simulink model "single_phase_afe"  (R2026b)
settings: Solver=ode23tb  StopTime=param.sim.simlength  FixedStep=param.sim.tc  MaxStep=param.glb_time.tc
values from neighbouring files (symbols this model uses):
  param = struct()    [init_model.m]
undefined symbols (not defined in the file or in its folder): magnitude
libraries: fl_lib x201, nesl_utility x108, igbt_simple_2th_lib x8, single_phase_pwm_modulator x2, dq_vector_pi x2, phase_shift_filter_ccaller x2, pi_ctrl x2, discrete_time_low_pass_filter x2, lithium_ion_battery x1, dclink_for_two_levels x1, three_phase_voltage_with_frt_emulator x1, simulink x1
(part 1 of 7)
settings Model: SimulationMode=accelerator  Creator=LTNBDA  LastModifiedBy=dbagn
settings SolverCC: AutoInsertRateTranBlk=on  SolverResetMethod=Robust  ZeroCrossAlgorithm=Adaptive  ZeroCrossControl=DisableAll
settings DataIOCC: DSMLogging=off  LimitDataPoints=on  MaxDataPoints=1  ReturnWorkspaceOutputs=off  SaveFormat=Array  SaveOutput=off  SaveTime=off  SignalLogging=off  SignalLoggingSaveFormat=ModelDataLogs
settings OptimizationCC: EfficientMapNaN2IntZero=off  LifeSpan=inf  MemsetInitFltsAndDblsToZero=off
settings DebuggingCC: ArithmeticOperatorsInVariantConditions=warning  FcnCallInpInsideContextMsg=warning  IgnoredZcDiagnostic=none  MergeDetectMultiDrivingBlocksExec=none  MultiTaskCondExecSysMsg=none  MultiTaskDSMMsg=warning  MultiTaskRateTransMsg=warning  SFNoUnconditionalDefaultTransitionDiag=warning  SFUnexpectedBacktrackingDiag=warning  SaveWithParameterizedLinksMsg=none  SignalResolutionControl=TryResolveAllWithWarning  SolverPrmCheckMsg=warning  StateNameClashWarn=warning
settings HardwareCC: ProdEndianess=Unspecified  ProdEqTarget=off  ProdHWDeviceType=Generic->64-bit Embedded Processor (LP64)  ProdIntDivRoundTo=Undefined  ProdLargestAtomicFloat=None  TargetEndianess=LittleEndian  TargetHWDeviceType=MATLAB Host  TargetIntDivRoundTo=Zero  TargetLongLongMode=on
settings ModelReferenceCC: PropagateSignalLabelsOutOfModel=off
settings SFSimCC: CustomCodeUndefinedFunction=UseInterfaceOnly  SimUseLocalCustomCode=off
settings SFSimCC: SimCustomHeaderCode=|
  | #include "phase_shift_flt_simulink.h"
  | #include "sv_pwm.h"
  | #include "rpi.h"
  | #include "rpi_simulink.h"
  | #include "first_harmonic_tracker.h"
  | #include "dqvector_pi.h"
  | #include "dqvector_pi_simulink.h"
  | #include "sv_pwm_simulink.h"
  | #include "dqpll_grid.h"
  | #include "first_harmonic_tracker_simulink.h"
  | #include "dqpll_grid_simulink.h"
  | #include "phase_shift_flt.h"
  | #include "math_f.h"
  | #include "linear_double_integrator_observer_simulink.h"
  | #include "linear_double_integrator_observer.h"
  | #include "sogi_flt_simulink.h"
  | #include "sogi_flt.h"
settings SFSimCC: SimUserIncludeDirs=|
  | include
  | src
settings SFSimCC: SimUserSources=|
  | "rpi.c"
  | "rpi_simulink.c"
  | "dqvector_pi_simulink.c"
  | "dqvector_pi.c"
  | "sv_pwm_simulink.c"
  | "sv_pwm.c"
  | "first_harmonic_tracker_simulink.c"
  | "first_harmonic_tracker.c"
  | "dqpll_grid_simulink.c"
  | "dqpll_grid.c"
  | "phase_shift_flt_simulink.c"
  | "phase_shift_flt.c"
  | "linear_double_integrator_observer_simulink.c"
  | "linear_double_integrator_observer.c"
  | "sogi_flt_simulink.c"
  | "sogi_flt.c"
settings RTWCC: RTWUseLocalCustomCode=off
settings CodeAppCC: StateflowObjectComments=on
settings GRTTargetCC: CombineOutputUpdateFcns=off  GRTInterface=on  TargetLangStandard=C89/C90 (ANSI)
settings ConfigComp: CovExternalEMLEnable=off  CovSaveCumulativeToWorkspaceVar=on  CovSaveSingleToWorkspaceVar=on
settings SimscapeCC: SimscapeNormalizeSystem=off  SimscapeUseEnergyAccounting=off

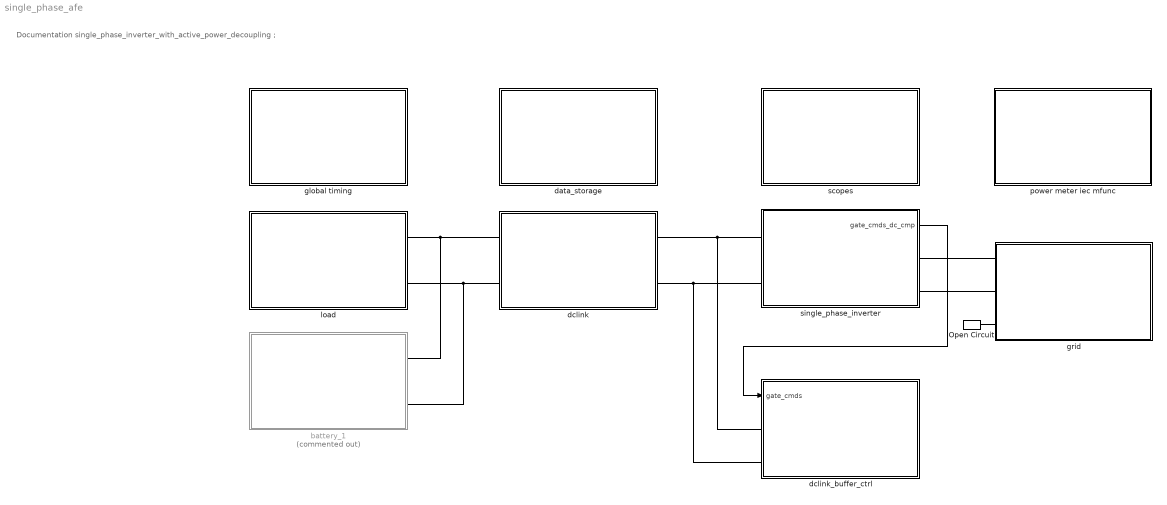
== system single_phase_afe ==
  note: Documentation
      | single_phase_inverter_with_active_power_decoupling ;
  Open Circuit : fl_lib/Electrical/Electrical Elements/Open Circuit  v_specify=off  v_priority=None  v=0 V  v_nominal_specify=off  v_nominal_value=1  v_nominal_unit=V
  battery_1 : Subsystem  Commented=on
  data_storage : Subsystem
  dclink : Subsystem
  dclink_buffer_ctrl : Subsystem
  global timing : Subsystem
  grid : Subsystem
  load : Subsystem
  power meter iec mfunc : Subsystem
  scopes : Subsystem
  single_phase_inverter : Subsystem
  wires:
  single_phase_inverter/1(gate_cmds_dc_cmp) -> dclink_buffer_ctrl/1(gate_cmds)
  connections:
  dclink/RConn2 -- dclink_buffer_ctrl/LConn2 -- single_phase_inverter/LConn2
  dclink/RConn1 -- dclink_buffer_ctrl/LConn1 -- single_phase_inverter/LConn1
  load/LConn2 -- battery_1/RConn2 -- dclink/LConn2
  load/LConn1 -- battery_1/RConn1 -- dclink/LConn1
  grid/RConn1 -- single_phase_inverter/RConn1
  grid/RConn2 -- single_phase_inverter/RConn2
  Open Circuit/LConn1 -- grid/RConn3

== system single_phase_afe/battery_1 ==
  To Workspace14 : ToWorkspace  VariableName=battery_1_data_sim  SampleTime=param.glb_time.tc
      settings: MaxDataPoints=param.glb_time.Nc  Decimation=param.glb_time.decimation_tc
  lithium ion battery : Scope
      settings: ActiveDisplayYMinimum=1112.6382819704118  ActiveDisplayYMaximum=1354.3206561925681  DataLoggingVariableName=ScopeData3
  lithium_ion_battery : lithium_ion_battery/lithium_ion_battery  Q=param.battery.pack_1.Q  number_of_cells=param.battery.pack_1.number_of_cells  E_1=param.battery.pack_1.E_1  E0=param.battery.pack_1.E0  E1=param.battery.pack_1.E1  E2=param.battery.pack_1.E2  E3=param.battery.pack_1.E3  Elog=param.battery.pack_1.Elog  R0=param.battery.pack_1.R0  R1=param.battery.pack_1.R1  C1=param.battery.pack_1.C1  M=param.battery.pack_1.M  alpha=param.battery.pack_1.alpha  soc_init=param.battery.pack_1.soc_init  ts_battery=param.glb_time.ts_dab  q1Kalman=param.battery.pack_1.q1Kalman  q2Kalman=param.battery.pack_1.q2Kalman  q3Kalman=param.battery.pack_1.q3Kalman  rKalman=param.battery.pack_1.rKalman  tc=param.glb_time.tc  enable_white_noise_m=0  battery_voltage_init_m=param.battery.nominal_battery_voltage_1
  single_phase_ui_measure : Subsystem
  dc(+) : PMIOPort  Side=Right
  dc(-) : PMIOPort  Port=2  Side=Right
  wires:
  lithium_ion_battery/1 -> To Workspace14/1, lithium ion battery/1
  connections:
  single_phase_ui_measure/LConn2 -- lithium_ion_battery/RConn2
  single_phase_ui_measure/RConn1 -- dc(+)/RConn1
  single_phase_ui_measure/LConn1 -- lithium_ion_battery/RConn1
  dc(-)/RConn1 -- single_phase_ui_measure/RConn2

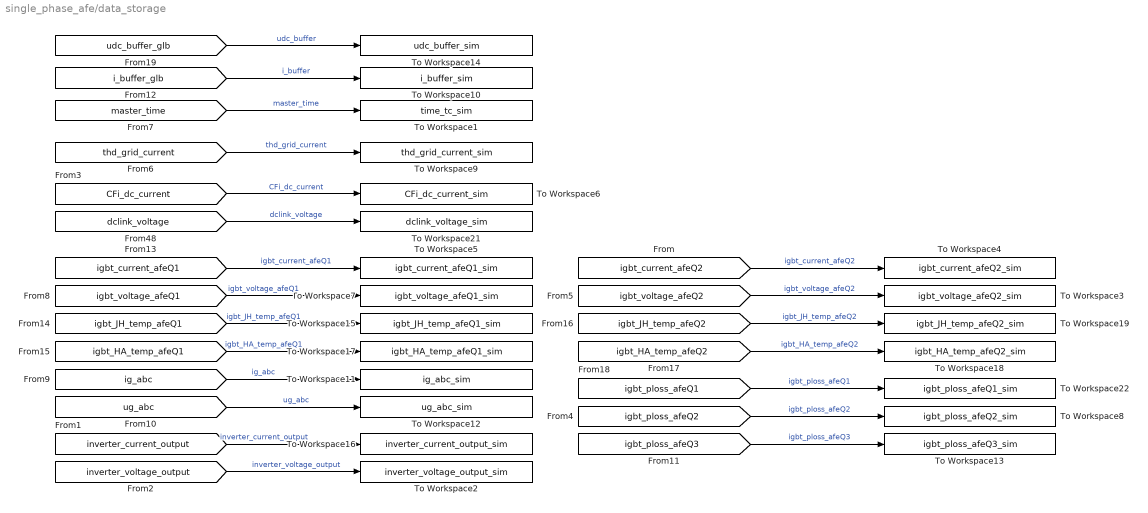
== system single_phase_afe/data_storage ==
  To Workspace1 : ToWorkspace  VariableName=time_tc_sim  SampleTime=param.glb_time.tc
      settings: MaxDataPoints=param.glb_time.Nc  Decimation=param.glb_time.decimation_tc
  To Workspace10 : ToWorkspace  VariableName=i_buffer_sim  SampleTime=param.glb_time.tc
      settings: MaxDataPoints=param.glb_time.Nc  Decimation=param.glb_time.decimation_tc
  To Workspace11 : ToWorkspace  VariableName=ig_abc_sim  SampleTime=param.glb_time.tc
      settings: MaxDataPoints=param.glb_time.Nc  Decimation=param.glb_time.decimation_tc
  To Workspace12 : ToWorkspace  VariableName=ug_abc_sim  SampleTime=param.glb_time.tc
      settings: MaxDataPoints=param.glb_time.Nc  Decimation=param.glb_time.decimation_tc
  To Workspace13 : ToWorkspace  VariableName=igbt_ploss_afeQ3_sim  SampleTime=param.glb_time.tc
      settings: MaxDataPoints=param.glb_time.Nc  Decimation=param.glb_time.decimation_tc
  To Workspace14 : ToWorkspace  VariableName=udc_buffer_sim  SampleTime=param.glb_time.tc
      settings: MaxDataPoints=param.glb_time.Nc  Decimation=param.glb_time.decimation_tc
  To Workspace15 : ToWorkspace  VariableName=igbt_JH_temp_afeQ1_sim  SampleTime=param.glb_time.tc
      settings: MaxDataPoints=param.glb_time.Nc  Decimation=param.glb_time.decimation_tc
  To Workspace16 : ToWorkspace  VariableName=inverter_current_output_sim  SampleTime=param.glb_time.tc
      settings: MaxDataPoints=param.glb_time.Nc  Decimation=param.glb_time.decimation_tc
  To Workspace17 : ToWorkspace  VariableName=igbt_HA_temp_afeQ1_sim  SampleTime=param.glb_time.tc
      settings: MaxDataPoints=param.glb_time.Nc  Decimation=param.glb_time.decimation_tc
  To Workspace18 : ToWorkspace  VariableName=igbt_HA_temp_afeQ2_sim  SampleTime=param.glb_time.tc
      settings: MaxDataPoints=param.glb_time.Nc  Decimation=param.glb_time.decimation_tc
  To Workspace19 : ToWorkspace  VariableName=igbt_JH_temp_afeQ2_sim  SampleTime=param.glb_time.tc
      settings: MaxDataPoints=param.glb_time.Nc  Decimation=param.glb_time.decimation_tc
  To Workspace2 : ToWorkspace  VariableName=inverter_voltage_output_sim  SampleTime=param.glb_time.tc
      settings: MaxDataPoints=param.glb_time.Nc  Decimation=param.glb_time.decimation_tc
  To Workspace21 : ToWorkspace  VariableName=dclink_voltage_sim  SampleTime=param.glb_time.tc
      settings: MaxDataPoints=param.glb_time.Nc  Decimation=param.glb_time.decimation_tc
  To Workspace22 : ToWorkspace  VariableName=igbt_ploss_afeQ1_sim  SampleTime=param.glb_time.tc
      settings: MaxDataPoints=param.glb_time.Nc  Decimation=param.glb_time.decimation_tc
  To Workspace3 : ToWorkspace  VariableName=igbt_voltage_afeQ2_sim  SampleTime=param.glb_time.tc
      settings: MaxDataPoints=param.glb_time.Nc  Decimation=param.glb_time.decimation_tc
  To Workspace4 : ToWorkspace  VariableName=igbt_current_afeQ2_sim  SampleTime=param.glb_time.tc
      settings: MaxDataPoints=param.glb_time.Nc  Decimation=param.glb_time.decimation_tc
  To Workspace5 : ToWorkspace  VariableName=igbt_current_afeQ1_sim  SampleTime=param.glb_time.tc
      settings: MaxDataPoints=param.glb_time.Nc  Decimation=param.glb_time.decimation_tc
  To Workspace6 : ToWorkspace  VariableName=CFi_dc_current_sim  SampleTime=param.glb_time.tc
      settings: MaxDataPoints=param.glb_time.Nc  Decimation=param.glb_time.decimation_tc
  To Workspace7 : ToWorkspace  VariableName=igbt_voltage_afeQ1_sim  SampleTime=param.glb_time.tc
      settings: MaxDataPoints=param.glb_time.Nc  Decimation=param.glb_time.decimation_tc
  To Workspace8 : ToWorkspace  VariableName=igbt_ploss_afeQ2_sim  SampleTime=param.glb_time.tc
      settings: MaxDataPoints=param.glb_time.Nc  Decimation=param.glb_time.decimation_tc
  To Workspace9 : ToWorkspace  VariableName=thd_grid_current_sim  SampleTime=param.glb_time.tc
      settings: MaxDataPoints=param.glb_time.Nc  Decimation=param.glb_time.decimation_tc
  wires:
  [inverter_current_output] -> To Workspace16/1  "inverter_current_output"
  [inverter_voltage_output] -> To Workspace2/1  "inverter_voltage_output"
  [CFi_dc_current] -> To Workspace6/1  "CFi_dc_current"
  [igbt_ploss_afeQ1] -> To Workspace22/1  "igbt_ploss_afeQ1"
  [dclink_voltage] -> To Workspace21/1  "dclink_voltage"
  [igbt_current_afeQ1] -> To Workspace5/1  "igbt_current_afeQ1"
  [igbt_voltage_afeQ2] -> To Workspace3/1  "igbt_voltage_afeQ2"
  [igbt_current_afeQ2] -> To Workspace4/1  "igbt_current_afeQ2"
  [igbt_voltage_afeQ1] -> To Workspace7/1  "igbt_voltage_afeQ1"
  [igbt_ploss_afeQ2] -> To Workspace8/1  "igbt_ploss_afeQ2"
  [ig_abc] -> To Workspace11/1  "ig_abc"
  [ug_abc] -> To Workspace12/1  "ug_abc"
  [igbt_JH_temp_afeQ1] -> To Workspace15/1  "igbt_JH_temp_afeQ1"
  [igbt_HA_temp_afeQ1] -> To Workspace17/1  "igbt_HA_temp_afeQ1"
  [igbt_JH_temp_afeQ2] -> To Workspace19/1  "igbt_JH_temp_afeQ2"
  [igbt_HA_temp_afeQ2] -> To Workspace18/1  "igbt_HA_temp_afeQ2"
  [igbt_ploss_afeQ3] -> To Workspace13/1  "igbt_ploss_afeQ3"
  [thd_grid_current] -> To Workspace9/1  "thd_grid_current"
  [master_time] -> To Workspace1/1  "master_time"
  [i_buffer_glb] -> To Workspace10/1  "i_buffer"
  [udc_buffer_glb] -> To Workspace14/1  "udc_buffer"

== system single_phase_afe/dclink ==
  dclink : dclink_for_two_levels/dclink  Cdc=param.afe.hw.CFi  Rudc_measure=1e6  Vdc_scale=param.afe.hw.udc_nom
  references : Subsystem
  Udc(+) : PMIOPort  Side=Right
  Udc(-) : PMIOPort  Port=2  Side=Right
  udc(+) : PMIOPort  Port=3  Side=Left
  udc(-) : PMIOPort  Port=4  Side=Left
  wires:
  dclink/1 -> references/1(m)
  connections:
  dclink/RConn1 -- udc(+)/RConn1
  dclink/RConn2 -- udc(-)/RConn1
  dclink/LConn1 -- Udc(+)/RConn1
  dclink/LConn2 -- Udc(-)/RConn1

== system single_phase_afe/dclink_buffer_ctrl ==
  gate_cmds : Inport
  Capacitor : fl_lib/Electrical/Electrical Elements/Capacitor  c=param.afe.buffer.C F  r=1e-6 Ohm  g=0 1/Ohm  i_specify=off  i_priority=None  i=0 A  i_nominal_specify=off  i_nominal_value=1  i_nominal_unit=A  v_specify=off  v_priority=None  v=0 V  v_nominal_specify=off  v_nominal_value=1  v_nominal_unit=V  vc_specify=off  vc_priority=High  vc=0 V  vc_nominal_specify=off  vc_nominal_value=1  vc_nominal_unit=V
  Current Sensor : fl_lib/Electrical/Electrical Sensors/Current Sensor
  Inductor : fl_lib/Electrical/Electrical Elements/Inductor  l=param.afe.buffer.L H  r=param.afe.buffer.RL Ohm  g=1e-9 1/Ohm  i_specify=off  i_priority=None  i=0 A  i_nominal_specify=off  i_nominal_value=1  i_nominal_unit=A  v_specify=off  v_priority=None  v=0 V  v_nominal_specify=off  v_nominal_value=1  v_nominal_unit=V  i_L_specify=off  i_L_priority=High  i_L=0 A  i_L_nominal_specify=off  i_L_nominal_value=1  i_L_nominal_unit=A
  Inductor1 : fl_lib/Electrical/Electrical Elements/Inductor  l=param.afe.buffer.L H  r=param.afe.buffer.RL Ohm  g=1e-9 1/Ohm  i_specify=off  i_priority=None  i=0 A  i_nominal_specify=off  i_nominal_value=1  i_nominal_unit=A  v_specify=off  v_priority=None  v=0 V  v_nominal_specify=off  v_nominal_value=1  v_nominal_unit=V  i_L_specify=off  i_L_priority=High  i_L=0 A  i_L_nominal_specify=off  i_L_nominal_value=1  i_L_nominal_unit=A
  PS-Simulink Converter : nesl_utility/PS-Simulink Converter  PhysicalDomain=network_engine_domain  SubClassName=ps_output  LeftPortType=input  RightPortType=output  PseudoPeriodic=off  Frequencies=[]  VectorFormat=1-D array  Unit=A  AffineConversion=off
  PS-Simulink Converter1 : nesl_utility/PS-Simulink Converter  PhysicalDomain=network_engine_domain  SubClassName=ps_output  LeftPortType=input  RightPortType=output  PseudoPeriodic=off  Frequencies=[]  VectorFormat=1-D array  Unit=V  AffineConversion=off
  Solver Configuration : nesl_utility/Solver Configuration  PhysicalDomain=network_engine_domain  SubClassName=solver  LeftPortType=input  RightPortType=generic  Tones=[]  Harmonics=[]  SimulateNoise=off  Profile=off  UseLocalSampling=off  EnableSwitchedLinearOptims=on  FrequencyDomain=off  UseCCode=off  RelTol=0.001  AbsTol=0.001  MinStep=1e-09  ToWorkspace=off  RevertToSquareIcSolve=off  NumHomotopyIterations=100  PhasorMode=off  PhasorModeNumHarmonics=1  ConsistencySolver=NEWTON_FTOL  CanonicalOrdering=UNORDERED  OptimizeIntermediates=UNOPTIMIZED  MulticoreSolverChoice=BACKWARD_EULER  IndexReductionMethod=DerivativeReplacement  DoDC=off  ResidualTolerance=1e-4  ConsistencyTolSource=GLOBAL  ConsistencyAbsTol=0.001  ConsistencyRelTol=0.001  ConsistencyTolFactor=0.001  UseLocalSolver=on  LocalSolverChoice=NE_BACKWARD_EULER_ADVANCER  ResolveIndetEquations=on  FunctionEvalNumThread=1  LocalSolverSampleTime=param.glb_time.tc  DoFixedCost=on  MaxNonlinIter=param.sim.nonlinear_iterations  MaxModeIter=2  ComputeImpulses=off  ImpulseIterations=2  LinearAlgebra=auto  LinearAlgebraNumThread=0  EquationFormulation=NE_TIME_EF  DelaysMemoryBudget=1024  AutomaticFiltering=on  FilteringTimeConstant=0.001  PartitionStorageMethod=AS_NEEDED  PartitionMemoryBudget=1024  PartitionMethod=BALANCED  MultibodyUseLocalSolver=off  MultibodyLocalSolverChoice=ODE1  MultibodyLocalSolverSampleTime=0.001
  Voltage Sensor : fl_lib/Electrical/Electrical Sensors/Voltage Sensor
  single_phase_inverter : Subsystem
  udc_buffer : Scope  NumInputPorts=3
      settings: ActiveDisplayString=3  ActiveDisplayYMinimum=431.30911748261815  ActiveDisplayYMaximum=2060.028861822575  DataLoggingVariableName=ScopeData16
  udc(+) : PMIOPort  Side=Left
  udc(-) : PMIOPort  Port=2  Side=Left
  tag scope: i_buffer_glb=global, udc_buffer_glb=global
  wires:
  gate_cmds/1 -> single_phase_inverter/1(gate_cmds)
  PS-Simulink Converter/1 -> [i_buffer_glb]
  PS-Simulink Converter1/1 -> [udc_buffer_glb], udc_buffer/1  "udc_buffer"
  [i_buffer_glb] -> udc_buffer/2  "i_buffer"
  [dclink_voltage] -> udc_buffer/3  "dclink_voltage"
  connections:
  Inductor1/RConn1 -- udc(-)/RConn1
  single_phase_inverter/RConn1 -- Inductor/RConn1
  single_phase_inverter/RConn2 -- Inductor1/LConn1
  Voltage Sensor/LConn1 -- Capacitor/LConn1 -- single_phase_inverter/LConn1
  Solver Configuration/RConn1 -- single_phase_inverter/LConn2 -- Voltage Sensor/RConn2 -- Capacitor/RConn1
  Current Sensor/RConn2 -- Inductor/LConn1
  udc(+)/RConn1 -- Current Sensor/LConn1
  Current Sensor/RConn1 -- PS-Simulink Converter/LConn1
  PS-Simulink Converter1/LConn1 -- Voltage Sensor/RConn1

== system single_phase_afe/global timing ==
  Unit Delay : UnitDelay  SampleTime=param.glb_time.tc
  time_afe1 : Subsystem  mask{k=1}
      mask prompts: k "Time Gain"
      mask Display:
      | disp('time-gen');
      | port_label('input', 1, 'crt');
      | port_label('output', 1, 'tout');
  time_afe3 : Subsystem  mask{k=1}
      mask prompts: k "Time Gain"
      mask Display:
      | disp('time-gen');
      | port_label('output', 1, 'tout');
  tag scope: master_time=global, time_afe_module_1=global
  wires:
  time_afe1/1(Out1) -> [time_afe_module_1]
  time_afe3/1(Out1) -> [master_time]
  Unit Delay/1 -> time_afe1/1(correction_time)

== system single_phase_afe/grid ==
  grid_emulator : Subsystem
  threephase_vi_measures : Subsystem
  ua : PMIOPort  Side=Right
  ub : PMIOPort  Port=2  Side=Right
  uc : PMIOPort  Port=3  Side=Right
  connections:
  threephase_vi_measures/LConn3 -- grid_emulator/RConn3
  threephase_vi_measures/LConn1 -- grid_emulator/RConn1
  threephase_vi_measures/RConn2 -- ub/RConn1
  threephase_vi_measures/LConn2 -- grid_emulator/RConn2
  threephase_vi_measures/RConn1 -- ua/RConn1
  threephase_vi_measures/RConn3 -- uc/RConn1

== system single_phase_afe/load ==
  load : fl_lib/Electrical/Electrical Elements/Resistor  Commented=on  R=param.load.R Ohm  i_specify=off  i_priority=None  i=0 A  i_nominal_specify=off  i_nominal_value=1  i_nominal_unit=A  v_specify=off  v_priority=None  v=0 V  v_nominal_specify=off  v_nominal_value=1  v_nominal_unit=V
  load_current_source : Subsystem
  udc(+) : PMIOPort  Side=Left
  udc(-) : PMIOPort  Port=2  Side=Left
  connections:
  load/RConn1 -- udc(-)/RConn1 -- load_current_source/RConn1
  udc(+)/RConn1 -- load_current_source/LConn1 -- load/LConn1

== system single_phase_afe/power meter iec mfunc ==
  Bus Selector : BusSelector  OutputSignals=Q1p,Q1n,P1n,P1p,U1n,U1p,i_act_1n,i_react_1n,i_act_1p,i_react_1p
  Constant : Constant  Value=param.glb_time.ts_afe
  Step : Step  Time=0.025  InitialValue=1  FinalValue=0  SampleTime=0
  To Workspace1 : ToWorkspace  VariableName=i_react_1n  SampleTime=param.glb_time.ts_afe
      settings: MaxDataPoints=param.glb_time.Ns_afe
  To Workspace2 : ToWorkspace  VariableName=i_react_1p  SampleTime=param.glb_time.ts_afe
      settings: MaxDataPoints=param.glb_time.Ns_afe
  To Workspace3 : ToWorkspace  VariableName=i_act_1n  SampleTime=param.glb_time.ts_afe
      settings: MaxDataPoints=param.glb_time.Ns_afe
  To Workspace4 : ToWorkspace  VariableName=i_act_1p  SampleTime=param.glb_time.ts_afe
      settings: MaxDataPoints=param.glb_time.Ns_afe
  To Workspace5 : ToWorkspace  VariableName=u1p  SampleTime=param.glb_time.ts_afe
      settings: MaxDataPoints=param.glb_time.Ns_afe
  To Workspace6 : ToWorkspace  VariableName=u1n  SampleTime=param.glb_time.ts_afe
      settings: MaxDataPoints=param.glb_time.Ns_afe
  Zero-Order Hold{,1..5} (6 alike) : ZeroOrderHold  SampleTime=param.glb_time.ts_afe
  three_phase_power_meter_iec : MATLAB Function  TreatAsAtomicUnit=on  SystemSampleTime=param.glb_time.ts_afe
  tag scope: P1n_global=global, P1p_global=global, Q1n_global=global, Q1p_global=global
  wires:
  Bus Selector/6 -> To Workspace5/1  "<U1p>"
  Bus Selector/8 -> To Workspace1/1  "<i_react_1n>"
  Bus Selector/10 -> To Workspace2/1  "<i_react_1p>"
  Bus Selector/5 -> To Workspace6/1  "<U1n>"
  Bus Selector/4 -> [P1p_global]  "<P1p>"
  Bus Selector/2 -> [Q1n_global]  "<Q1n>"
  Bus Selector/1 -> [Q1p_global]  "<Q1p>"
  Bus Selector/7 -> To Workspace3/1  "<i_act_1n>"
  Bus Selector/9 -> To Workspace4/1  "<i_act_1p>"
  Bus Selector/3 -> [P1n_global]  "<P1n>"
  three_phase_power_meter_iec/1(m) -> Bus Selector/1
  Zero-Order Hold/1 -> three_phase_power_meter_iec/1(phase)
  Zero-Order Hold2/1 -> three_phase_power_meter_iec/3(i_abc)
  [phase_grid_emulator] -> Zero-Order Hold/1
  Step/1 -> Zero-Order Hold5/1
  Zero-Order Hold3/1 -> three_phase_power_meter_iec/4(omega)
  Zero-Order Hold4/1 -> three_phase_power_meter_iec/5(ts)
  [ug_abc] -> Zero-Order Hold1/1
  Zero-Order Hold5/1 -> three_phase_power_meter_iec/6(enable_time)
  [ig_abc] -> Zero-Order Hold2/1
  [pulsation_grid_emulator] -> Zero-Order Hold3/1
  Constant/1 -> Zero-Order Hold4/1
  Zero-Order Hold1/1 -> three_phase_power_meter_iec/2(u_abc)

== system single_phase_afe/scopes ==
  Bus Creator : BusCreator  Inputs=2
  Bus Creator1 : BusCreator  Inputs=3
  Bus Creator2 : BusCreator  Inputs=2
  THD : Subsystem
  global_ctrl_performance : Scope  NumInputPorts=4
      settings: ActiveDisplayYMinimum=-5267.1431025743714  ActiveDisplayYMaximum=7950.1528448964045
  grid power meter : Scope  NumInputPorts=4
      settings: ActiveDisplayString=3  ActiveDisplayYMinimum=-68573.869128089456  ActiveDisplayYMaximum=92300.8379469249  DataLoggingVariableName=ScopeData4
  ig_abc/ug_abc : Scope  NumInputPorts=2
      settings: SampleTime=param.glb_time.tc  ActiveDisplayYMinimum=-728.98568173233309  ActiveDisplayYMaximum=715.77264260288678  DataLoggingVariableName=ScopeData5
  igbt_current_voltage : Scope  NumInputPorts=2
      settings: SampleTime=param.glb_time.tc  ActiveDisplayYMinimum=-268.04135278991151  ActiveDisplayYMaximum=2412.3721564377493  DataLoggingVariableName=ScopeData7
  inverter current/voltage output : Scope  NumInputPorts=2
      settings: ActiveDisplayYMinimum=-1688.705418622251  ActiveDisplayYMaximum=2229.3684372465282
  power_loss mosfet_inv : Scope  NumInputPorts=2
      settings: SampleTime=param.glb_time.tc  ActiveDisplayYMinimum=-186.67737399665268  ActiveDisplayYMaximum=1680.0963659698743  DataLoggingVariableName=ScopeData6
  tag scope: thd_grid_current=global
  wires:
  [dclink_voltage] -> global_ctrl_performance/3  "dclink_voltage"
  [i_buffer_glb] -> global_ctrl_performance/2  "dclink_buffer_current"
  [ug_abc] -> ig_abc/ug_abc/2  "vg_abc"
  [ig_abc] -> ig_abc/ug_abc/1  "ig_abc"
  [igbt_ploss_afeQ1] -> power_loss mosfet_inv/1  "igbt_ploss_afeQ1"
  [igbt_JH_temp_afeQ1] -> Bus Creator/1  "igbt_JH_temp_afeQ1"
  [igbt_HA_temp_afeQ1] -> Bus Creator/2  "igbt_HA_temp_afeQ1"
  Bus Creator/1 -> power_loss mosfet_inv/2
  [igbt_current_afeQ1] -> igbt_current_voltage/1  "igbt_current_afeQ1"
  [igbt_voltage_afeQ1] -> igbt_current_voltage/2  "igbt_voltage_afeQ1"
  [dclink_voltage] -> Bus Creator1/1  "dclink_voltage"
  [dclink_p2gnd_voltage] -> Bus Creator1/2  "dclink_p2gnd_voltage"
  [dclink_n2gnd_voltage] -> Bus Creator1/3  "dclink_n2gnd_voltage"
  [Q1p_global] -> grid power meter/1  "Q1p_global"
  [Q1n_global] -> grid power meter/2  "Q1n_global"
  [P1n_global] -> grid power meter/3  "P1n_global"
  [P1p_global] -> grid power meter/4  "P1p_global"
  Bus Creator1/1 -> inverter current/voltage output/1
  [ig_mod1] -> Bus Creator2/2, THD/1(signal)  "grid_current"
  [inverter_current_output] -> Bus Creator2/1  "inverter_output_current"
  Bus Creator2/1 -> inverter current/voltage output/2, global_ctrl_performance/1
  THD/1(thd_pct) -> [thd_grid_current], global_ctrl_performance/4  "thd_grid_current"

== system single_phase_afe/single_phase_inverter ==
  grid_filter : Subsystem
  single phase inverter control : Subsystem
  single_phase_inverter : Subsystem
  vi_measures_grid : Subsystem
  uac(+) : PMIOPort  Side=Right
  uac(-) : PMIOPort  Port=2  Side=Right
  udc(+) : PMIOPort  Port=3  Side=Left
  udc(-) : PMIOPort  Port=4  Side=Left
  gate_cmds_dc_cmp : Outport
  wires:
  single phase inverter control/2(gate_cmds) -> single_phase_inverter/1(gate_cmds)
  single phase inverter control/1(gate_cmds_dc_comp) -> gate_cmds_dc_cmp/1
  connections:
  single_phase_inverter/LConn1 -- udc(+)/RConn1
  single_phase_inverter/LConn2 -- udc(-)/RConn1
  vi_measures_grid/RConn1 -- uac(+)/RConn1
  vi_measures_grid/RConn2 -- uac(-)/RConn1
  single_phase_inverter/RConn1 -- grid_filter/LConn1
  vi_measures_grid/LConn1 -- grid_filter/RConn1
  single_phase_inverter/RConn2 -- grid_filter/LConn2
  vi_measures_grid/LConn2 -- grid_filter/RConn2

== system single_phase_afe/battery_1/single_phase_ui_measure ==
  Bus Creator : BusCreator  Inputs=2
  Current Sensor : fl_lib/Electrical/Electrical Sensors/Current Sensor
  Selector : Selector  InputPortWidth=2  IndexOptions=Index vector (dialog)  Indices=2  OutputSizes=1  RuntimeRangeChecks=off
  Selector1 : Selector  InputPortWidth=2  IndexOptions=Index vector (dialog)  Indices=1  OutputSizes=1  RuntimeRangeChecks=off
  Voltage Sensor : fl_lib/Electrical/Electrical Sensors/Voltage Sensor
  dab input modA : Scope  NumInputPorts=2
      settings: SampleTime=param.glb_time.tc  ActiveDisplayYMinimum=-596.930724759566  ActiveDisplayYMaximum=217.35258636886869  DataLoggingVariableName=ScopeData2
  iph : nesl_utility/PS-Simulink Converter  PhysicalDomain=network_engine_domain  SubClassName=ps_output  LeftPortType=input  RightPortType=output  PseudoPeriodic=off  Frequencies=[]  VectorFormat=1-D array  Unit=A  AffineConversion=off
  uph : nesl_utility/PS-Simulink Converter  PhysicalDomain=network_engine_domain  SubClassName=ps_output  LeftPortType=input  RightPortType=output  PseudoPeriodic=off  Frequencies=[]  VectorFormat=1-D array  Unit=V  AffineConversion=off
  Udc(+) : PMIOPort  Side=Left
  udc(+) : PMIOPort  Port=2  Side=Right
  Udc(-) : PMIOPort  Port=3  Side=Left
  udc(-) : PMIOPort  Port=4  Side=Right
  tag scope: current_battery_1=global, voltage_battery_1=global
  wires:
  Bus Creator/1 -> Selector/1, Selector1/1  "ui_data"
  iph/1 -> Bus Creator/1  "iph"
  uph/1 -> Bus Creator/2  "uph"
  Selector1/1 -> [current_battery_1], dab input modA/1  "current_battery"
  Selector/1 -> dab input modA/2, [voltage_battery_1]  "voltage_battery"
  connections:
  iph/LConn1 -- Current Sensor/RConn1
  Voltage Sensor/LConn1 -- Current Sensor/LConn1 -- Udc(+)/RConn1
  Current Sensor/RConn2 -- udc(+)/RConn1
  Voltage Sensor/RConn1 -- uph/LConn1
  Voltage Sensor/RConn2 -- Udc(-)/RConn1 -- udc(-)/RConn1

== system single_phase_afe/dclink/references ==
  m : Inport
  Bus Selector : BusSelector  OutputSignals=udc,udc_p_gnd,udc_n_gnd,Cdc1_current
  tag scope: CFi_dc_current=global, dclink_n2gnd_voltage=global, dclink_p2gnd_voltage=global, dclink_voltage=global
  wires:
  m/1 -> Bus Selector/1
  Bus Selector/1 -> [dclink_voltage]  "<udc>"
  Bus Selector/4 -> [CFi_dc_current]  "<Cdc1_current>"
  Bus Selector/3 -> [dclink_n2gnd_voltage]  "<udc_n_gnd>"
  Bus Selector/2 -> [dclink_p2gnd_voltage]  "<udc_p_gnd>"

== system single_phase_afe/dclink_buffer_ctrl/single_phase_inverter ==
  gate_cmds : Inport
  single phase inverter : Subsystem
      settings: PortSchema="{\"entries\":[{\"content\":{\"sides\":[{\"content\":{\"connectorIds\":[\"LConn1\",\"LConn2\"]},\"type\":\"ConnectorPlacement.EquallySpacedRectSide\",\"uuid\":\"4fcf4fea-d38f-431b-8a91-be3ce9782faf\"},{\"content\":{\"connectorIds\":[\"RConn1\",\"RConn2\"],\"side\":\"RIGHT\"},\"type\":\"ConnectorPlacement.EquallySpacedRectSide\",\"uuid\":\"0aa56277-92e9-4e3b-84c7-43398254a4d8\"},{\"content\":{\"connectorIds\":[\"In1\"],\"side\":\"TOP\"},\"type\":\"ConnectorPlacement.EquallySpacedRectSide\",\"uuid\":\"5cd150dc-bcaf-4cd7-b2a8-3db203726730\"}]},\"type\":\"ConnectorPlacement.EquallySpacedConnector\",\"uuid\":\"bf8194c4-c327-4d40-bea4-f1e7617f80b4\"}],\"packageUris\":[\"http://schema.mathworks.com/mf0/Connector/R2020b\"],\"version\":\"1.0\"}"
  uac(+) : PMIOPort  Side=Right
  uac(-) : PMIOPort  Port=2  Side=Right
  udc(+) : PMIOPort  Port=3  Side=Left
  udc(-) : PMIOPort  Port=4  Side=Left
  wires:
  gate_cmds/1 -> single phase inverter/1(gate_cmds)
  connections:
  single phase inverter/RConn1 -- udc(+)/RConn1
  single phase inverter/LConn2 -- uac(-)/RConn1
  uac(+)/RConn1 -- single phase inverter/LConn1
  single phase inverter/RConn2 -- udc(-)/RConn1

== system single_phase_afe/global timing/time_afe1 ==
  correction_time : Inport
  Constant : Constant
  Gain : Gain  Gain=k
  Product : Product
  Sum : Sum  Inputs=|++
  time_1 : Clock
  Out1 : Outport
  wires:
  time_1/1 -> Gain/1
  Gain/1 -> Product/1
  Product/1 -> Out1/1
  correction_time/1 -> Sum/1
  Sum/1 -> Product/2
  Constant/1 -> Sum/2

== system single_phase_afe/global timing/time_afe3 ==
  Gain : Gain  Gain=k
  time_1 : Clock
  Out1 : Outport
  wires:
  Gain/1 -> Out1/1
  time_1/1 -> Gain/1

== system single_phase_afe/grid/grid_emulator ==
  Bus Selector : BusSelector  OutputSignals=ua_grid_emu,ub_grid_emu,uc_grid_emu
  Bus Selector1 : BusSelector  OutputSignals=gamma_grid_emulator,omega_grid_emulator
  Controlled Voltage Source : fl_lib/Electrical/Electrical Sources/Controlled Voltage Source
  Controlled Voltage Source1 : fl_lib/Electrical/Electrical Sources/Controlled Voltage Source
  Controlled Voltage Source2 : fl_lib/Electrical/Electrical Sources/Controlled Voltage Source
  Electrical Reference : fl_lib/Electrical/Electrical Elements/Electrical Reference
  Simulink-PS Converter : nesl_utility/Simulink-PS Converter  PhysicalDomain=network_engine_domain  SubClassName=ps_input  LeftPortType=input  RightPortType=output  PseudoPeriodic=off  Frequencies=[]  NoiseDistribution=none  NoiseParameters=[]  Unit=V  AffineConversion=on  FilteringAndDerivatives=provide  SimscapeFilterOrder=1  InputFilterTimeConstant=0.001  UdotUserProvided=0
  Simulink-PS Converter1 : nesl_utility/Simulink-PS Converter  PhysicalDomain=network_engine_domain  SubClassName=ps_input  LeftPortType=input  RightPortType=output  PseudoPeriodic=off  Frequencies=[]  NoiseDistribution=none  NoiseParameters=[]  Unit=V  AffineConversion=on  FilteringAndDerivatives=provide  SimscapeFilterOrder=1  InputFilterTimeConstant=0.001  UdotUserProvided=0
  Simulink-PS Converter2 : nesl_utility/Simulink-PS Converter  PhysicalDomain=network_engine_domain  SubClassName=ps_input  LeftPortType=input  RightPortType=output  PseudoPeriodic=off  Frequencies=[]  NoiseDistribution=none  NoiseParameters=[]  Unit=V  AffineConversion=on  FilteringAndDerivatives=provide  SimscapeFilterOrder=1  InputFilterTimeConstant=0.001  UdotUserProvided=0
  three_phase_voltage_source_with_frt_emulator : three_phase_voltage_with_frt_emulator/three_phase_voltage_source_with_frt_emulator  nominal_frequency_m=param.grid.emu.fgrid_nom  nominal_voltage_m=param.grid.emu.us_nom  Vemu_ref_norm_m=param.grid.emu.Vemu_ref_norm  vp_xi_pu_m=param.grid.emu.up_xi_pu_ref  vp_eta_pu_m=param.grid.emu.up_eta_pu_ref  vn_xi_pu_m=param.grid.emu.un_xi_pu_ref  vn_eta_pu_m=param.grid.emu.un_eta_pu_ref  Am=param.grid.emu.sof_50Hz.A  Bm=param.grid.emu.sof_50Hz.B  Cm=param.grid.emu.sof_50Hz.C  enable_frt_1_m=param.grid.frt.enable_frt_1  enable_frt_2_m=param.grid.frt.enable_frt_2  start_time_LVRT_m=param.grid.frt.start_time_LVRT  end_time_LVRT_m=param.grid.frt.end_time_LVRT  deepPOSxi_m=param.grid.frt.deepPOSxi  deepPOSeta_m=param.grid.frt.deepPOSeta  deepNEGxi_m=param.grid.frt.deepNEGxi  deepNEGeta_m=param.grid.frt.deepNEGeta  Amplitude_U_m=param.grid.frt.Amplitude_U  Amplitude_V_m=param.grid.frt.Amplitude_V  Amplitude_W_m=param.grid.frt.Amplitude_W  t_ramp_m=param.grid.frt.t_ramp  Phase_shift_m=param.grid.frt.Phase_shift
  threephase_vi_measures : Subsystem
  u1 : PMIOPort  Side=Right
  u2 : PMIOPort  Port=2  Side=Right
  u3 : PMIOPort  Port=3  Side=Right
  tag scope: phase_grid_emulator=global, pulsation_grid_emulator=global
  wires:
  Bus Selector1/2 -> [pulsation_grid_emulator]  "<omega_grid_emulator>"
  Bus Selector1/1 -> [phase_grid_emulator]  "<gamma_grid_emulator>"
  Bus Selector/2 -> Simulink-PS Converter1/1  "<ub_grid_emu>"
  Bus Selector/3 -> Simulink-PS Converter2/1  "<uc_grid_emu>"
  three_phase_voltage_source_with_frt_emulator/1 -> Bus Selector1/1, Bus Selector/1
  Bus Selector/1 -> Simulink-PS Converter/1  "<ua_grid_emu>"
  connections:
  Simulink-PS Converter/RConn1 -- Controlled Voltage Source/RConn1
  Simulink-PS Converter1/RConn1 -- Controlled Voltage Source1/RConn1
  Simulink-PS Converter2/RConn1 -- Controlled Voltage Source2/RConn1
  Controlled Voltage Source/RConn2 -- Controlled Voltage Source1/RConn2 -- Electrical Reference/LConn1 -- Controlled Voltage Source2/RConn2
  u1/RConn1 -- threephase_vi_measures/RConn1
  u2/RConn1 -- threephase_vi_measures/RConn2
  u3/RConn1 -- threephase_vi_measures/RConn3
  Controlled Voltage Source/LConn1 -- threephase_vi_measures/LConn1
  Controlled Voltage Source1/LConn1 -- threephase_vi_measures/LConn2
  Controlled Voltage Source2/LConn1 -- threephase_vi_measures/LConn3

== system single_phase_afe/grid/threephase_vi_measures ==
  Bus Creator : BusCreator  Inputs=6
  Current Sensor : fl_lib/Electrical/Electrical Sensors/Current Sensor
  Current Sensor1 : fl_lib/Electrical/Electrical Sensors/Current Sensor
  Current Sensor2 : fl_lib/Electrical/Electrical Sensors/Current Sensor
  Electrical Reference1 : fl_lib/Electrical/Electrical Elements/Electrical Reference
  Selector : Selector  InputPortWidth=6  IndexOptions=Index vector (dialog)  Indices=[1 2 3]  OutputSizes=1  RuntimeRangeChecks=off
  Selector1 : Selector  InputPortWidth=6  IndexOptions=Index vector (dialog)  Indices=[4 5 6]  OutputSizes=1  RuntimeRangeChecks=off
  Voltage Sensor : fl_lib/Electrical/Electrical Sensors/Voltage Sensor
  Voltage Sensor1 : fl_lib/Electrical/Electrical Sensors/Voltage Sensor
  Voltage Sensor2 : fl_lib/Electrical/Electrical Sensors/Voltage Sensor
  ia_grid : nesl_utility/PS-Simulink Converter  PhysicalDomain=network_engine_domain  SubClassName=ps_output  LeftPortType=input  RightPortType=output  PseudoPeriodic=off  Frequencies=[]  VectorFormat=1-D array  Unit=A  AffineConversion=off
  ib_grid : nesl_utility/PS-Simulink Converter  PhysicalDomain=network_engine_domain  SubClassName=ps_output  LeftPortType=input  RightPortType=output  PseudoPeriodic=off  Frequencies=[]  VectorFormat=1-D array  Unit=A  AffineConversion=off
  ic_grid : nesl_utility/PS-Simulink Converter  PhysicalDomain=network_engine_domain  SubClassName=ps_output  LeftPortType=input  RightPortType=output  PseudoPeriodic=off  Frequencies=[]  VectorFormat=1-D array  Unit=A  AffineConversion=off
  ig_abc/ug_abc : Scope  NumInputPorts=2
      settings: SampleTime=param.glb_time.tc  ActiveDisplayYMinimum=-662.618491750231  ActiveDisplayYMaximum=662.00821995187164  DataLoggingVariableName=ScopeData2
  ua_grid : nesl_utility/PS-Simulink Converter  PhysicalDomain=network_engine_domain  SubClassName=ps_output  LeftPortType=input  RightPortType=output  PseudoPeriodic=off  Frequencies=[]  VectorFormat=1-D array  Unit=V  AffineConversion=off
  ub_grid : nesl_utility/PS-Simulink Converter  PhysicalDomain=network_engine_domain  SubClassName=ps_output  LeftPortType=input  RightPortType=output  PseudoPeriodic=off  Frequencies=[]  VectorFormat=1-D array  Unit=V  AffineConversion=off
  uc_grid : nesl_utility/PS-Simulink Converter  PhysicalDomain=network_engine_domain  SubClassName=ps_output  LeftPortType=input  RightPortType=output  PseudoPeriodic=off  Frequencies=[]  VectorFormat=1-D array  Unit=V  AffineConversion=off
  Ua : PMIOPort  Side=Left
  ua : PMIOPort  Port=2  Side=Right
  Ub : PMIOPort  Port=3  Side=Left
  ub : PMIOPort  Port=4  Side=Right
  Uc : PMIOPort  Port=5  Side=Left
  uc : PMIOPort  Port=6  Side=Right
  tag scope: ig_abc=global, ug_abc=global
  wires:
  Bus Creator/1 -> Selector1/1, Selector/1  "vi_data"
  Selector/1 -> [ug_abc]
  ib_grid/1 -> Bus Creator/5  "ib"
  ia_grid/1 -> Bus Creator/4  "ia"
  ic_grid/1 -> Bus Creator/6  "ic"
  ua_grid/1 -> Bus Creator/1  "ua"
  ub_grid/1 -> Bus Creator/2  "ub"
  uc_grid/1 -> Bus Creator/3  "uc"
  Selector1/1 -> [ig_abc]
  [ug_abc] -> ig_abc/ug_abc/2  "ug_abc(line)"
  [ig_abc] -> ig_abc/ug_abc/1  "ig_abc(line)"
  connections:
  Current Sensor1/LConn1 -- Ub/RConn1 -- Voltage Sensor1/LConn1
  Electrical Reference1/LConn1 -- Voltage Sensor/RConn2 -- Voltage Sensor2/RConn2 -- Voltage Sensor1/RConn2
  Voltage Sensor/RConn1 -- ua_grid/LConn1
  Current Sensor/RConn2 -- ua/RConn1
  Voltage Sensor1/RConn1 -- ub_grid/LConn1
  Voltage Sensor2/LConn1 -- Current Sensor2/LConn1 -- Uc/RConn1
  Current Sensor/LConn1 -- Ua/RConn1 -- Voltage Sensor/LConn1
  Current Sensor1/RConn2 -- ub/RConn1
  Voltage Sensor2/RConn1 -- uc_grid/LConn1
  ib_grid/LConn1 -- Current Sensor1/RConn1
  ia_grid/LConn1 -- Current Sensor/RConn1
  ic_grid/LConn1 -- Current Sensor2/RConn1
  Current Sensor2/RConn2 -- uc/RConn1

== system single_phase_afe/load/load_current_source ==
  PS Ramp : fl_lib/Physical Signals/Sources/PS Ramp  slope=param.load.i_slope 1/s  start_time=0 s  initial_output=0  ZeroCross=true
  PS Saturation : fl_lib/Physical Signals/Nonlinear Operators/PS Saturation  upper_limit=param.load.i_max  lower_limit=-param.load.i_max  ZeroCross=true
  load_current : fl_lib/Electrical/Electrical Sources/Controlled Current Source
  udc(+) : PMIOPort  Side=Left
  udc(-) : PMIOPort  Port=2  Side=Right
  connections:
  PS Ramp/RConn1 -- PS Saturation/LConn1
  PS Saturation/RConn1 -- load_current/RConn1
  udc(+)/RConn1 -- load_current/LConn1
  udc(-)/RConn1 -- load_current/RConn2

== system single_phase_afe/scopes/THD ==
  signal : Inport
  Constant : Constant  Value=1/param.glb_time.tc
  Constant1 : Constant  Value=25
  Constant2 : Constant  Value=200e-3/param.glb_time.tc
  Constant3 : Constant  Value=10e-3/param.glb_time.tc
  Data Type Conversion : DataTypeConversion  OutDataTypeStr=int32  SaturateOnIntegerOverflow=off  RndMeth=Floor
  Data Type Conversion1 : DataTypeConversion  OutDataTypeStr=int32  SaturateOnIntegerOverflow=off  RndMeth=Floor
  Data Type Conversion2 : DataTypeConversion  OutDataTypeStr=int32  SaturateOnIntegerOverflow=off  RndMeth=Floor
  Scope : Scope  NumInputPorts=3
      settings: ActiveDisplayYMinimum=0.20306614530530309  ActiveDisplayYMaximum=12.861474899934214  DataLoggingVariableName=ScopeData14
  thd : MATLAB Function  TreatAsAtomicUnit=on  SystemSampleTime=param.glb_time.tc
  thd_pct : Outport
  wires:
  Constant3/1 -> Data Type Conversion1/1
  signal/1 -> thd/1(u)
  Constant2/1 -> Data Type Conversion/1
  thd/1(thd_pct) -> Scope/1, thd_pct/1
  Constant1/1 -> Data Type Conversion2/1
  thd/2(f1) -> Scope/2
  thd/3(valid) -> Scope/3
  Constant/1 -> thd/2(fs)
  Data Type Conversion/1 -> thd/4(N)
  Data Type Conversion1/1 -> thd/5(Nupd)
  Data Type Conversion2/1 -> thd/3(nHarm)

== system single_phase_afe/single_phase_inverter/grid_filter ==
  CFu : fl_lib/Electrical/Electrical Elements/Capacitor  c=param.afe.hw.CFu F  r=param.afe.hw.RCFu Ohm  g=0 1/Ohm  i_specify=off  i_priority=None  i=0 A  i_nominal_specify=off  i_nominal_value=1  i_nominal_unit=A  v_specify=off  v_priority=None  v=0 V  v_nominal_specify=off  v_nominal_value=1  v_nominal_unit=V  vc_specify=off  vc_priority=High  vc=0 V  vc_nominal_specify=off  vc_nominal_value=1  vc_nominal_unit=V
  LFu1 : fl_lib/Electrical/Electrical Elements/Inductor  l=param.afe.hw.LFu1 H  r=param.afe.hw.RLFu1 Ohm  g=1e-9 1/Ohm  i_specify=on  i_priority=High  i=0 A  i_nominal_specify=off  i_nominal_value=1  i_nominal_unit=A  v_specify=off  v_priority=None  v=0 V  v_nominal_specify=off  v_nominal_value=1  v_nominal_unit=V  i_L_specify=off  i_L_priority=High  i_L=0 A  i_L_nominal_specify=off  i_L_nominal_value=1  i_L_nominal_unit=A
  LFu2 : fl_lib/Electrical/Electrical Elements/Inductor  l=param.afe.hw.LFu2 H  r=param.afe.hw.RLFu2 Ohm  g=1e-9 1/Ohm  i_specify=on  i_priority=High  i=0 A  i_nominal_specify=off  i_nominal_value=1  i_nominal_unit=A  v_specify=off  v_priority=None  v=0 V  v_nominal_specify=off  v_nominal_value=1  v_nominal_unit=V  i_L_specify=off  i_L_priority=High  i_L=0 A  i_L_nominal_specify=off  i_L_nominal_value=1  i_L_nominal_unit=A
  Uac(+) : PMIOPort  Side=Left
  uac(+) : PMIOPort  Port=2  Side=Right
  Uac(-) : PMIOPort  Port=3  Side=Left
  uac(-) : PMIOPort  Port=4  Side=Right
  connections:
  LFu2/RConn1 -- uac(-)/RConn1 -- CFu/RConn1
  LFu1/RConn1 -- uac(+)/RConn1 -- CFu/LConn1
  Uac(-)/RConn1 -- LFu2/LConn1
  Uac(+)/RConn1 -- LFu1/LConn1

== system single_phase_afe/single_phase_inverter/single phase inverter control ==
  acquisition_and_scaling_current_buffer : Subsystem
  acquisition_and_scaling_current_with_white_noise : Subsystem
  acquisition_and_scaling_dc_voltage : Subsystem
  acquisition_and_scaling_dc_voltage_buffer : Subsystem
  acquisition_and_scaling_grid_voltage_ac : Subsystem
  acquisition_and_scaling_voltage : Subsystem
  grid_phase_hat_performance : Scope  NumInputPorts=2
  pwm modulator : Subsystem
  pwm modulator_dclink_compensator : Subsystem
  single_phase_inverter_ctrl : Subsystem
  gate_cmds_dc_comp : Outport
  gate_cmds : Outport  Port=2
  wires:
  [inverter_current_output] -> acquisition_and_scaling_current_with_white_noise/1(in)
  pwm modulator/1(gate_cmds) -> gate_cmds/1
  [TRGO_AFE_1] -> single_phase_inverter_ctrl/Trigger
  [inverter_voltage_output] -> acquisition_and_scaling_voltage/1(in)
  single_phase_inverter_ctrl/1(u_ctrl_out) -> pwm modulator/1(vout)
  acquisition_and_scaling_current_with_white_noise/1(out) -> single_phase_inverter_ctrl/2(inverter_current_output_pu)  "inverter_current_output_pu"
  acquisition_and_scaling_voltage/1(out) -> single_phase_inverter_ctrl/1(inverter_voltage_output_pu)  "inverter_voltage_output_pu"
  [dclink_voltage] -> acquisition_and_scaling_dc_voltage/1(in)
  acquisition_and_scaling_dc_voltage/1(out) -> single_phase_inverter_ctrl/3(dclink_voltage_pu)  "dclink_voltage_pu"
  [time_afe_module_1] -> single_phase_inverter_ctrl/4(local_time)
  [ug_abc] -> acquisition_and_scaling_grid_voltage_ac/1(in)
  acquisition_and_scaling_grid_voltage_ac/1(out) -> single_phase_inverter_ctrl/5(ugrid_pu)  "ug_abc"
  single_phase_inverter_ctrl/3(grid_phase_hat) -> grid_phase_hat_performance/1  "grid_phase_hat"
  [phase_grid_emulator] -> grid_phase_hat_performance/2
  [i_buffer_glb] -> acquisition_and_scaling_current_buffer/1(in)
  acquisition_and_scaling_current_buffer/1(out) -> single_phase_inverter_ctrl/6(i_buffer_pu)
  pwm modulator_dclink_compensator/1(gate_cmds) -> gate_cmds_dc_comp/1
  single_phase_inverter_ctrl/2(u_ctrl_buffer) -> pwm modulator_dclink_compensator/1(vout)
  [udc_buffer_glb] -> acquisition_and_scaling_dc_voltage_buffer/1(in)
  acquisition_and_scaling_dc_voltage_buffer/1(out) -> single_phase_inverter_ctrl/7(udc_buffer_pu)

== system single_phase_afe/single_phase_inverter/single_phase_inverter ==
  gate_cmds : Inport
  Current Sensor : fl_lib/Electrical/Electrical Sensors/Current Sensor
  Voltage Sensor1 : fl_lib/Electrical/Electrical Sensors/Voltage Sensor
  iph : nesl_utility/PS-Simulink Converter  PhysicalDomain=network_engine_domain  SubClassName=ps_output  LeftPortType=input  RightPortType=output  PseudoPeriodic=off  Frequencies=[]  VectorFormat=1-D array  Unit=A  AffineConversion=off
  single phase inverter : Subsystem
      settings: PortSchema="{\"entries\":[{\"content\":{\"sides\":[{\"content\":{\"connectorIds\":[\"LConn1\",\"LConn2\"]},\"type\":\"ConnectorPlacement.EquallySpacedRectSide\",\"uuid\":\"4fcf4fea-d38f-431b-8a91-be3ce9782faf\"},{\"content\":{\"connectorIds\":[\"RConn1\",\"RConn2\"],\"side\":\"RIGHT\"},\"type\":\"ConnectorPlacement.EquallySpacedRectSide\",\"uuid\":\"0aa56277-92e9-4e3b-84c7-43398254a4d8\"},{\"content\":{\"connectorIds\":[\"In1\"],\"side\":\"TOP\"},\"type\":\"ConnectorPlacement.EquallySpacedRectSide\",\"uuid\":\"5cd150dc-bcaf-4cd7-b2a8-3db203726730\"}]},\"type\":\"ConnectorPlacement.EquallySpacedConnector\",\"uuid\":\"bf8194c4-c327-4d40-bea4-f1e7617f80b4\"}],\"packageUris\":[\"http://schema.mathworks.com/mf0/Connector/R2020b\"],\"version\":\"1.0\"}"
  uph1 : nesl_utility/PS-Simulink Converter  PhysicalDomain=network_engine_domain  SubClassName=ps_output  LeftPortType=input  RightPortType=output  PseudoPeriodic=off  Frequencies=[]  VectorFormat=1-D array  Unit=V  AffineConversion=off
  uac(+) : PMIOPort  Side=Right
  uac(-) : PMIOPort  Port=2  Side=Right
  udc(+) : PMIOPort  Port=3  Side=Left
  udc(-) : PMIOPort  Port=4  Side=Left
  tag scope: inverter_current_output=global, inverter_voltage_output=global
  wires:
  iph/1 -> [inverter_current_output]  "inverter_current_output"
  uph1/1 -> [inverter_voltage_output]  "inverter_voltage_output"
  gate_cmds/1 -> single phase inverter/1(gate_cmds)
  connections:
  Current Sensor/RConn2 -- uac(+)/RConn1 -- Voltage Sensor1/LConn1
  single phase inverter/RConn1 -- udc(+)/RConn1
  iph/LConn1 -- Current Sensor/RConn1
  single phase inverter/LConn2 -- uac(-)/RConn1 -- Voltage Sensor1/RConn2
  Voltage Sensor1/RConn1 -- uph1/LConn1
  single phase inverter/LConn1 -- Current Sensor/LConn1
  single phase inverter/RConn2 -- udc(-)/RConn1

== system single_phase_afe/single_phase_inverter/vi_measures_grid ==
  Current Sensor : fl_lib/Electrical/Electrical Sensors/Current Sensor
  Gain1 : Gain  Gain=1/param.grid.emu.u2bez
  Gain6 : Gain  Gain=1/param.afe.hw.ibez
  Voltage Sensor : fl_lib/Electrical/Electrical Sensors/Voltage Sensor
  ia_grid : nesl_utility/PS-Simulink Converter  PhysicalDomain=network_engine_domain  SubClassName=ps_output  LeftPortType=input  RightPortType=output  PseudoPeriodic=off  Frequencies=[]  VectorFormat=1-D array  Unit=A  AffineConversion=off
  ua_grid : nesl_utility/PS-Simulink Converter  PhysicalDomain=network_engine_domain  SubClassName=ps_output  LeftPortType=input  RightPortType=output  PseudoPeriodic=off  Frequencies=[]  VectorFormat=1-D array  Unit=V  AffineConversion=off
  Uac(+) : PMIOPort  Side=Left
  uac(+) : PMIOPort  Port=2  Side=Right
  Uac(-) : PMIOPort  Port=3  Side=Left
  uac(-) : PMIOPort  Port=4  Side=Right
  tag scope: ig_mod1=global, ig_pu_mod1=global, ug_mod1=global, ug_pu_mod1=global
  wires:
  ua_grid/1 -> [ug_mod1], Gain1/1
  ia_grid/1 -> [ig_mod1], Gain6/1
  Gain1/1 -> [ug_pu_mod1]  "ua_grid_pu"
  Gain6/1 -> [ig_pu_mod1]  "ia_grid_pu"
  connections:
  ia_grid/LConn1 -- Current Sensor/RConn1
  Voltage Sensor/LConn1 -- Current Sensor/LConn1 -- Uac(+)/RConn1
  Current Sensor/RConn2 -- uac(+)/RConn1
  Voltage Sensor/RConn1 -- ua_grid/LConn1
  Voltage Sensor/RConn2 -- uac(-)/RConn1 -- Uac(-)/RConn1

== system single_phase_afe/dclink_buffer_ctrl/single_phase_inverter/single phase inverter ==
  gate_cmds : Inport
  three_phase_inverter_with_igbt_simple_2th : Subsystem
  uac_out(+) : PMIOPort  Side=Left
  uac_out(-) : PMIOPort  Port=2  Side=Left
  udc(+) : PMIOPort  Port=3  Side=Right
  udc(-) : PMIOPort  Port=4  Side=Right
  wires:
  gate_cmds/1 -> three_phase_inverter_with_igbt_simple_2th/1(gate_cmds)
  connections:
  udc(-)/RConn1 -- three_phase_inverter_with_igbt_simple_2th/LConn2
  udc(+)/RConn1 -- three_phase_inverter_with_igbt_simple_2th/LConn1
  uac_out(+)/RConn1 -- three_phase_inverter_with_igbt_simple_2th/RConn1
  uac_out(-)/RConn1 -- three_phase_inverter_with_igbt_simple_2th/RConn2
